simulink model "industrial_dc_motor_drive_control"  (R2024b)
settings: Solver=VariableStepAuto  StartTime=0.0  StopTime=15  RelTol=1e-3
libraries: fl_lib x11, nesl_utility x5, slpidlib x1
settings Model: Creator=Taha  LastModifiedBy=Taha

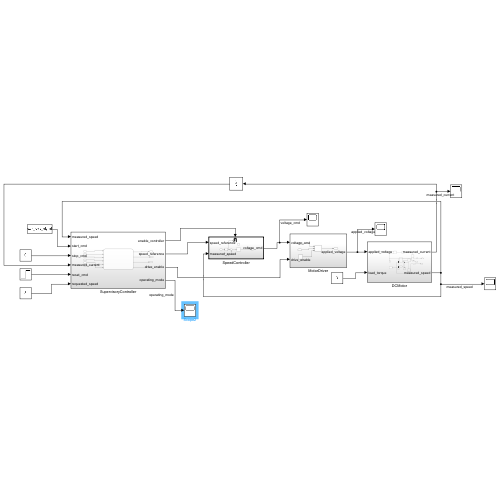
[thumbnail: Simulink's stored preview of the top-level diagram]
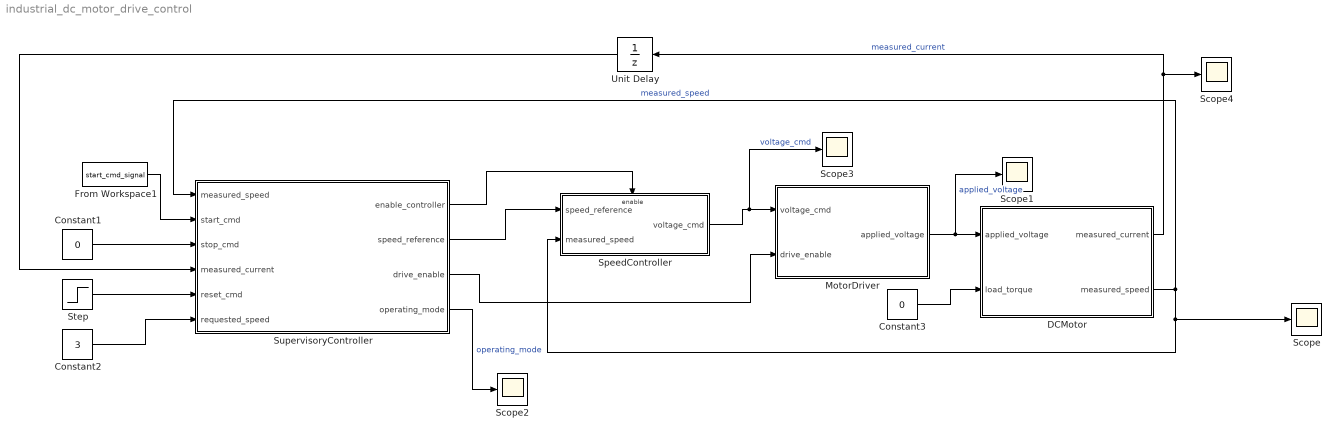
== system industrial_dc_motor_drive_control ==
  Constant1 : Constant  Value=0
  Constant2 : Constant  Value=3
  Constant3 : Constant  Value=0
  DCMotor : Subsystem
  From Workspace1 : FromWorkspace  VariableName=start_cmd_signal  Interpolate=off  OutputAfterFinalValue=Holding final value
  MotorDriver : Subsystem
  Scope{,1..4} (5 alike) : Scope
  SpeedController : Subsystem  TreatAsAtomicUnit=on
  Step : Step  Time=10  SampleTime=0
  SupervisoryController : Subsystem
  Unit Delay : UnitDelay  SampleTime=0.01  HasFrameUpgradeWarning=on
  wires:
  MotorDriver/1(applied_voltage) -> Scope1/1, DCMotor/1(applied_voltage)  "applied_voltage"
  SpeedController/1(voltage_cmd) -> Scope3/1, MotorDriver/1(voltage_cmd)  "voltage_cmd"
  DCMotor/2(measured_speed) -> Scope/1, SpeedController/2(measured_speed), SupervisoryController/1(measured_speed)  "measured_speed"
  DCMotor/1(measured_current) -> Scope4/1, Unit Delay/1  "measured_current"
  SupervisoryController/2(speed_reference) -> SpeedController/1(speed_reference)
  SupervisoryController/3(drive_enable) -> MotorDriver/2(drive_enable)
  From Workspace1/1 -> SupervisoryController/2(start_cmd)
  Constant1/1 -> SupervisoryController/3(stop_cmd)
  Step/1 -> SupervisoryController/5(reset_cmd)
  Constant2/1 -> SupervisoryController/6(requested_speed)
  Constant3/1 -> DCMotor/2(load_torque)
  SupervisoryController/1(enable_controller) -> SpeedController/Enable
  SupervisoryController/4(operating_mode) -> Scope2/1  "operating_mode"
  Unit Delay/1 -> SupervisoryController/4(measured_current)

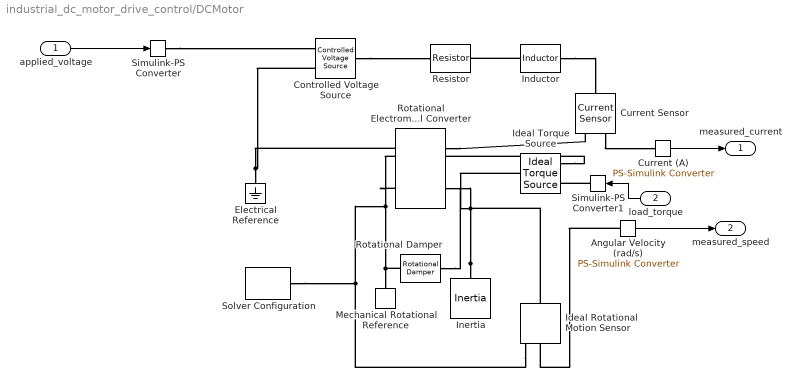
== system industrial_dc_motor_drive_control/DCMotor ==
  applied_voltage : Inport
  load_torque : Inport  Port=2
  Angular Velocity (rad/s) : nesl_utility/PS-Simulink Converter  PhysicalDomain=network_engine_domain  SubClassName=ps_output  LeftPortType=input  RightPortType=output  PseudoPeriodic=off  Frequencies=[]  VectorFormat=inherit  Unit=rad/s  AffineConversion=off
  Controlled Voltage Source : fl_lib/Electrical/Electrical Sources/Controlled Voltage Source
  Current (A) : nesl_utility/PS-Simulink Converter  PhysicalDomain=network_engine_domain  SubClassName=ps_output  LeftPortType=input  RightPortType=output  PseudoPeriodic=off  Frequencies=[]  VectorFormat=inherit  Unit=A  AffineConversion=off
  Current Sensor : fl_lib/Electrical/Electrical Sensors/Current Sensor
  Electrical Reference : fl_lib/Electrical/Electrical Elements/Electrical Reference
  Ideal Rotational Motion Sensor : fl_lib/Mechanical/Mechanical Sensors/Ideal Rotational Motion Sensor  reference=foundation.enum.MeasurementReference.difference  acceleration_port=false  velocity_port=true  position_port=true  wrap_angle=false  offset=0 rad
  Ideal Torque Source : fl_lib/Mechanical/Mechanical Sources/Ideal Torque Source
  Inductor : fl_lib/Electrical/Electrical Elements/Inductor  l=0.5 H  r=0 Ohm  g=1e-9 1/Ohm  i_specify=off  i_priority=None  i=0 A  i_nominal_specify=off  i_nominal_value=1  i_nominal_unit=A  v_specify=off  v_priority=None  v=0 V  v_nominal_specify=off  v_nominal_value=1  v_nominal_unit=V  i_L_specify=off  i_L_priority=High  i_L=0 A  i_L_nominal_specify=off  i_L_nominal_value=1  i_L_nominal_unit=A
  Inertia : fl_lib/Mechanical/Rotational Elements/Inertia  inertia=0.01 kg*m^2  num_ports=foundation.enum.numPorts2.one  w_specify=off  w_priority=High  w=0 rad/s  w_nominal_specify=off  w_nominal_value=1  w_nominal_unit=rad/s  t_specify=off  t_priority=None  t=0 N*m  t_nominal_specify=off  t_nominal_value=1  t_nominal_unit=N*m
  Mechanical Rotational Reference : fl_lib/Mechanical/Rotational Elements/Mechanical Rotational Reference
  Resistor : fl_lib/Electrical/Electrical Elements/Resistor  R=1 Ohm  i_specify=off  i_priority=None  i=0 A  i_nominal_specify=off  i_nominal_value=1  i_nominal_unit=A  v_specify=off  v_priority=None  v=0 V  v_nominal_specify=off  v_nominal_value=1  v_nominal_unit=V
  Rotational Electromechanical Converter : fl_lib/Electrical/Electrical Elements/Rotational Electromechanical Converter  K=0.01 V*s/rad  i_specify=off  i_priority=None  i=0 A  i_nominal_specify=off  i_nominal_value=1  i_nominal_unit=A  v_specify=off  v_priority=None  v=0 V  v_nominal_specify=off  v_nominal_value=1  v_nominal_unit=V  t_specify=off  t_priority=None  t=0 N*m  t_nominal_specify=off  t_nominal_value=1  t_nominal_unit=N*m  w_specify=off  w_priority=None  w=0 rad/s  w_nominal_specify=off  w_nominal_value=1  w_nominal_unit=rad/s
  Rotational Damper : fl_lib/Mechanical/Rotational Elements/Rotational Damper  D=0.1 N*m*s/rad  w_specify=off  w_priority=None  w=0 rad/s  w_nominal_specify=off  w_nominal_value=1  w_nominal_unit=rad/s  t_specify=off  t_priority=None  t=0 N*m  t_nominal_specify=off  t_nominal_value=1  t_nominal_unit=N*m
  Simulink-PS Converter : nesl_utility/Simulink-PS Converter  PhysicalDomain=network_engine_domain  SubClassName=ps_input  LeftPortType=input  RightPortType=output  PseudoPeriodic=off  Frequencies=[]  NoiseDistribution=none  NoiseParameters=[]  Unit=1  AffineConversion=off  FilteringAndDerivatives=provide  SimscapeFilterOrder=1  InputFilterTimeConstant=0.001  UdotUserProvided=0
  Simulink-PS Converter1 : nesl_utility/Simulink-PS Converter  PhysicalDomain=network_engine_domain  SubClassName=ps_input  LeftPortType=input  RightPortType=output  PseudoPeriodic=off  Frequencies=[]  NoiseDistribution=none  NoiseParameters=[]  Unit=N*m  AffineConversion=off  FilteringAndDerivatives=provide  SimscapeFilterOrder=1  InputFilterTimeConstant=0.001  UdotUserProvided=0
  Solver Configuration : nesl_utility/Solver Configuration  PhysicalDomain=network_engine_domain  SubClassName=solver  LeftPortType=input  RightPortType=generic  Tones=[]  Harmonics=[]  SimulateNoise=off  Profile=off  UseLocalSampling=off  EnableSwitchedLinearOptims=on  FrequencyDomain=off  UseCCode=off  RelTol=0.001  AbsTol=1e-06  MinStep=1e-09  ToWorkspace=off  RevertToSquareIcSolve=off  NumHomotopyIterations=100  PhasorMode=off  PhasorModeNumHarmonics=1  ConsistencySolver=NEWTON_XTOL_AFTER_FTOL  IndexReductionMethod=DerivativeReplacement  DoDC=off  ResidualTolerance=1e-09  ConsistencyTolSource=GLOBAL  ConsistencyAbsTol=0.001  ConsistencyRelTol=0.001  ConsistencyTolFactor=0.001  UseLocalSolver=off  LocalSolverChoice=NE_BACKWARD_EULER_ADVANCER  ResolveIndetEquations=on  FunctionEvalNumThread=1  LocalSolverSampleTime=0.001  DoFixedCost=off  MaxNonlinIter=3  MaxModeIter=2  ComputeImpulses=off  ImpulseIterations=2  LinearAlgebra=auto  LinearAlgebraNumThread=0  EquationFormulation=NE_TIME_EF  DelaysMemoryBudget=1024  AutomaticFiltering=on  FilteringTimeConstant=0.001  PartitionStorageMethod=AS_NEEDED  PartitionMemoryBudget=1024  PartitionMethod=ROBUST  MultibodyUseLocalSolver=off  MultibodyLocalSolverChoice=ODE1  MultibodyLocalSolverSampleTime=0.001
  measured_current : Outport
  measured_speed : Outport  Port=2
  wires:
  load_torque/1 -> Simulink-PS Converter1/1
  applied_voltage/1 -> Simulink-PS Converter/1
  Current (A)/1 -> measured_current/1
  Angular Velocity (rad/s)/1 -> measured_speed/1
  connections:
  Solver Configuration/RConn1 -- Rotational Electromechanical Converter/RConn2 -- Ideal Torque Source/RConn2 -- Rotational Damper/RConn1 -- Mechanical Rotational Reference/LConn1 -- Ideal Rotational Motion Sensor/RConn1
  Inertia/LConn1 -- Rotational Electromechanical Converter/LConn2 -- Rotational Damper/LConn1 -- Ideal Torque Source/LConn1 -- Ideal Rotational Motion Sensor/LConn1
  Electrical Reference/LConn1 -- Rotational Electromechanical Converter/RConn1 -- Controlled Voltage Source/RConn2
  Angular Velocity (rad/s)/LConn1 -- Ideal Rotational Motion Sensor/RConn2
  Inductor/LConn1 -- Resistor/RConn1
  Controlled Voltage Source/LConn1 -- Resistor/LConn1
  Simulink-PS Converter/RConn1 -- Controlled Voltage Source/RConn1
  Rotational Electromechanical Converter/LConn1 -- Current Sensor/RConn2
  Inductor/RConn1 -- Current Sensor/LConn1
  Simulink-PS Converter1/RConn1 -- Ideal Torque Source/RConn1
  Current Sensor/RConn1 -- Current (A)/LConn1

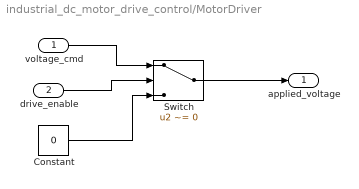
== system industrial_dc_motor_drive_control/MotorDriver ==
  voltage_cmd : Inport
  drive_enable : Inport  Port=2
  Constant : Constant  Value=0
  Switch : Switch  Criteria=u2 ~= 0  SaturateOnIntegerOverflow=off  InputSameDT=off
  applied_voltage : Outport
  wires:
  Switch/1 -> applied_voltage/1
  voltage_cmd/1 -> Switch/1
  drive_enable/1 -> Switch/2
  Constant/1 -> Switch/3

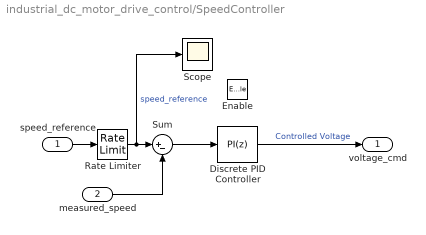
== system industrial_dc_motor_drive_control/SpeedController ==
  speed_reference : Inport
  measured_speed : Inport  Port=2
  Enable : EnablePort
  Discrete PID Controller : slpidlib/PID Controller  Controller=PI  Form=Parallel  TimeDomain=Discrete-time  UseExternalTs=off  SampleTime=0.01  IntegratorMethod=Forward Euler  FilterMethod=Forward Euler  ControllerParametersSource=internal  P=16.579207  I=35  UseKiTs=off  D=0  UseExternalDerivativeSource=off  N=100  UseFilter=on  TunerSelectOption=Transfer Function Based (PID Tuner App)  InitialConditionSource=internal  InitialConditionForIntegrator=0  InitialConditionForFilter=0  DifferentiatorICPrevScaledInput=0  ExternalReset=none  TrackingMode=off  Kt=1  LimitOutput=on  SatLimitsSource=internal  UpperSaturationLimit=120  LowerSaturationLimit=-120  LinearizeAsGain=off  AntiWindupMode=clamping  Kb=1  LimitIntegrator=off  UpperIntegratorSaturationLimit=inf  LowerIntegratorSaturationLimit=-inf  POutMin=[]  POutMax=[]  IOutMin=[]  IOutMax=[]  DOutMin=[]  DOutMax=[]  NOutMin=[]  NOutMax=[]  SumOutMin=[]  SumOutMax=[]  SaturationOutMin=[]  SaturationOutMax=[]  PParamMin=[]  PParamMax=[]  IParamMin=[]  IParamMax=[]  DParamMin=[]  DParamMax=[]  NParamMin=[]  NParamMax=[]  KbParamMin=[]  KbParamMax=[]  KtParamMin=[]  KtParamMax=[]  KbOutMin=[]  KbOutMax=[]  KtOutMin=[]  KtOutMax=[]  IntegratorOutMin=[]  IntegratorOutMax=[]  FilterOutMin=[]  FilterOutMax=[]  SumI1OutMin=[]  SumI1OutMax=[]  SumI2OutMin=[]  SumI2OutMax=[]  SumI3OutMin=[]  SumI3OutMax=[]  SumI4OutMin=[]  SumI4OutMax=[]  SumDOutMin=[]  SumDOutMax=[]  DifferentiatorOutMin=[]  DifferentiatorOutMax=[]  FilterDiffOutCoefMin=[]  FilterDiffOutCoefMax=[]  ReciprocalOutMin=[]  ReciprocalOutMax=[]  SumDenOutMin=[]  SumDenOutMax=[]  SumNumOutMin=[]  SumNumOutMax=[]  DivideOutMin=[]  DivideOutMax=[]  UdiffTsProdOutMin=[]  UdiffTsProdOutMax=[]  NTsProdOutMin=[]  NTsProdOutMax=[]  UintegralTsProdOutMin=[]  UintegralTsProdOutMax=[]  UngainTsProdOutMin=[]  UngainTsProdOutMax=[]  ClampingZeroOutDataTypeStr=Inherit: Inherit via back propagation  ClampingZeroOutMin=[]  ClampingZeroOutMax=[]  FilterDenConstantOutDataTypeStr=Inherit: Inherit via back propagation  FilterDenConstantOutMin=[]  FilterDenConstantOutMax=[]  PCopyOutDataTypeStr=Inherit: Inherit via back propagation  PCopyOutMin=[]  PCopyOutMax=[]  NCopyOutDataTypeStr=Inherit: Inherit via back propagation  NCopyOutMin=[]  NCopyOutMax=[]  IntegratorContinuousStateAttributes=''  IntegratorStateMustResolveToSignalObject=off  IntegratorRTWStateStorageClass=Auto  FilterContinuousStateAttributes=''  FilterStateMustResolveToSignalObject=off  FilterRTWStateStorageClass=Auto  ParallelPVariant=InternalParameters  IdealPVariant=Disabled  IVariant=InternalParameters  DVariant=Disabled  IntegratorVariant=Discrete  SatVariant=Enabled  AWVariant=DiscClampingParallel  PCopyVariant=Disabled  TRVariant=Disabled  FdbkBlocksVariant=Forward  IdealPFdbkVariant=Disabled  SatFdbkVariant=Disabled  DerivativeFilterVariant=Disabled  NVariant=Disabled  NCopyVariant=Disabled_SignalSpec  FilterICVariant=Disabled  IntegratorICVariant=InternalICs  ExternalResetVariant=Disabled  TRSumVariant=Passthrough  SumFdbkVariant=Disabled  SumVariant=Sum_PI  TsampFilterVariant=InternalTs  TsampNgainVariant=Passthrough  TsampIntegralVariant=Disabled_SignalSpec  ExternalSaturationOutDataTypeStr=Inherit: Same as second input  DerivativeSourceVariant=Disabled  PreIntVariant=InternalPreInt
      settings: LibrarySourceBlock=simulink/Discrete/Discrete PID Controller
  Rate Limiter : RateLimiter  RisingSlewLimit=0.5  FallingSlewLimit=-0.5  SampleTimeMode=inherited
  Scope : Scope
  Sum : Sum  Inputs=|+-
  voltage_cmd : Outport
  wires:
  Sum/1 -> Discrete PID Controller/1
  Discrete PID Controller/1 -> voltage_cmd/1  "Controlled Voltage"
  speed_reference/1 -> Rate Limiter/1
  measured_speed/1 -> Sum/2
  Rate Limiter/1 -> Scope/1, Sum/1  "speed_reference"

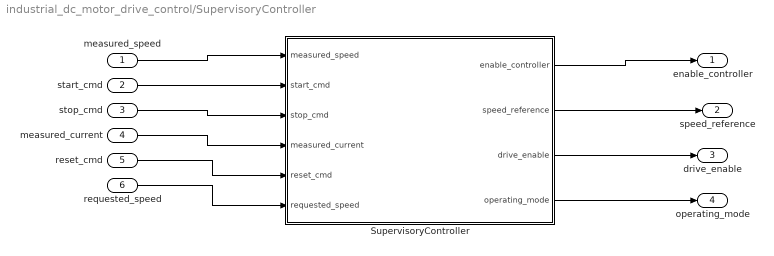
== system industrial_dc_motor_drive_control/SupervisoryController ==
  measured_speed : Inport
  start_cmd : Inport  Port=2
  stop_cmd : Inport  Port=3
  measured_current : Inport  Port=4
  reset_cmd : Inport  Port=5
  requested_speed : Inport  Port=6
  SupervisoryController : Stateflow chart  TreatAsAtomicUnit=on
  enable_controller : Outport
  speed_reference : Outport  Port=2
  drive_enable : Outport  Port=3
  operating_mode : Outport  Port=4
  wires:
  measured_speed/1 -> SupervisoryController/1(measured_speed)
  start_cmd/1 -> SupervisoryController/2(start_cmd)
  stop_cmd/1 -> SupervisoryController/3(stop_cmd)
  measured_current/1 -> SupervisoryController/4(measured_current)
  reset_cmd/1 -> SupervisoryController/5(reset_cmd)
  requested_speed/1 -> SupervisoryController/6(requested_speed)
  SupervisoryController/4(operating_mode) -> operating_mode/1
  SupervisoryController/2(speed_reference) -> speed_reference/1
  SupervisoryController/3(drive_enable) -> drive_enable/1
  SupervisoryController/1(enable_controller) -> enable_controller/1

== stateflow chart industrial_dc_motor_drive_control/SupervisoryController/SupervisoryController ==
  settings: updateMethod=DISCRETE  sampleTime=0.01
  state IDLE
    entry:
    enable_controller = false;
    drive_enable = false;
    speed_reference = 0;
    operating_mode = uint8(0);
  state RUNNING
    entry:
    enable_controller = true;
    drive_enable = true;
    speed_reference = requested_speed;
    operating_mode = uint8(1);
    during:
    speed_reference = requested_speed;
  state STOPPING
    entry:
    enable_controller = true;
    drive_enable = true;
    speed_reference = 0;
    operating_mode = uint8(2);
  state FAULT
    entry:
    enable_controller = false;
    drive_enable = false;
    speed_reference = 0;
    operating_mode = uint8(3);
  (default) -> IDLE
  IDLE -> RUNNING [order 2] : [hasChangedTo(start_cmd, 1) && abs(measured_current) <= current_limit && ~stop_cmd]
  RUNNING -> STOPPING [order 2] : [stop_cmd]
  FAULT -> IDLE : [reset_cmd && abs(measured_current) <= current_limit && ~start_cmd]
  IDLE -> FAULT [order 1] : [abs(measured_current) > current_limit]
  STOPPING -> IDLE [order 2] : [abs(measured_speed) < speed_tolerance]
  RUNNING -> FAULT [order 1] : [abs(measured_current) > current_limit]
  STOPPING -> FAULT [order 1] : [abs(measured_current) > current_limit]
  data: measured_speed input; start_cmd input; stop_cmd input; speed_tolerance local =0.02; measured_current input; current_limit local =20; reset_cmd input; enable_controller output boolean; speed_reference output double; drive_enable output boolean; operating_mode output uint8; requested_speed input double
